simulink model "A2_live"  (R2024b)
settings: Solver=ode4  StartTime=0.0  StopTime=T_run  FixedStep=Ts_ctrl  RelTol=1e-3
values from neighbouring files (symbols this model uses):
  animate = 1    [A2_6_gps_setup.m]    (also in A2_gui_setup.m; A2_live_setup.m)
  R_LOS = evalin('base', 'R_LOS')    [A2_gui_report.m]
  Ts_ctrl = evalin('base', 'Ts_ctrl')    [A2_gui_report.m]
  u_ref = evalin('base', 'u_ref')    [A2_gui_report.m]
  wp_east = wp_ned(:,2).'    [A2_3_click_done.m]    (also in A2_3_click_todo.m; A2_6_gps_setup.m = [0   15   60   35]; A2_gui_report.m = evalin('base', 'wp_east'); A2_gui_setup.m = zeros(1, WP_MAX))
  wp_north = wp_ned(:,1).'    [A2_3_click_done.m]    (also in A2_3_click_todo.m; A2_6_gps_setup.m = [0   30   30   -5]; A2_gui_report.m = evalin('base', 'wp_north'); A2_gui_setup.m = zeros(1, WP_MAX))
  x0 = [0.1; 0; 0; 0; 0; psi_init]    [A2_6_gps_setup.m]    (also in A2_gui_setup.m = [0.1; 0; 0; 0; 0; 0]; A2_live_setup.m)
undefined symbols (not defined in the file or in its folder): beta_c, current_speed, Delta, F_max, F_plugin_max, guidance_mode, half_beam, k_prop, Kb, Kd_psi, Ki_u, Kp_psi, Kp_u, stop_hold, sw_mode, usv_p
libraries: slpidlib x1
settings Model: Creator=admin  LastModifiedBy=admin

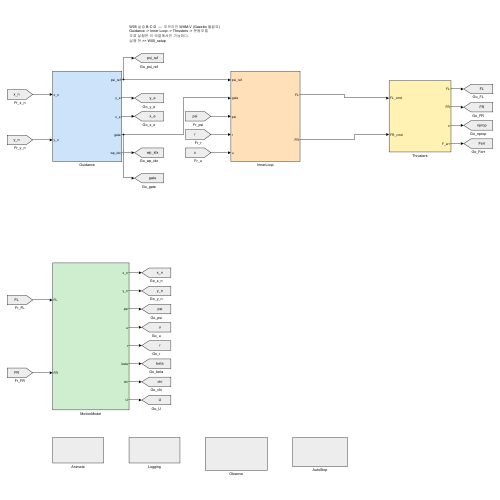
[thumbnail: Simulink's stored preview of the top-level diagram]
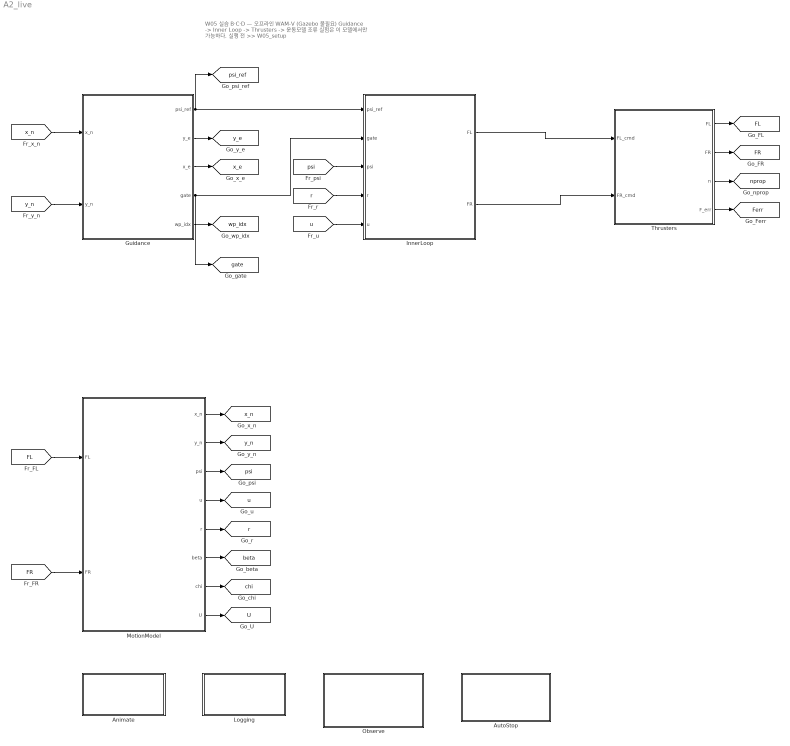
== system A2_live ==
  note: W05 실습 B·C·D  —  오프라인 WAM-V (Gazebo 불필요)
      | Guidance -> Inner Loop -> Thrusters -> 운동모델
      | 조류 실험은 이 모델에서만 가능하다.
      | 실행 전 >> W05_setup
  Animate : Subsystem
  AutoStop : Subsystem
  Guidance : Subsystem
  InnerLoop : Subsystem
  Logging : Subsystem
  MotionModel : Subsystem
  Observe : Subsystem
  Thrusters : Subsystem
  tag scope: FL=global, FR=global, Ferr=global, U=global, beta=global, chi=global, gate=global, nprop=global, psi=global, psi_ref=global, r=global, u=global, wp_idx=global, x_e=global, x_n=global, y_e=global, y_n=global
  wires:
  InnerLoop/2(FR) -> Thrusters/2(FR_cmd)
  InnerLoop/1(FL) -> Thrusters/1(FL_cmd)
  Guidance/4(gate) -> InnerLoop/2(gate), [gate]
  Guidance/1(psi_ref) -> InnerLoop/1(psi_ref), [psi_ref]
  Thrusters/1(FL) -> [FL]
  Thrusters/2(FR) -> [FR]
  Thrusters/3(n) -> [nprop]
  MotionModel/3(psi) -> [psi]
  MotionModel/5(r) -> [r]
  MotionModel/4(u) -> [u]
  MotionModel/1(x_n) -> [x_n]
  Guidance/2(y_e) -> [y_e]
  MotionModel/2(y_n) -> [y_n]
  [FL] -> MotionModel/1(FL)
  [FR] -> MotionModel/2(FR)
  [psi] -> InnerLoop/3(psi)
  [r] -> InnerLoop/4(r)
  [u] -> InnerLoop/5(u)
  [x_n] -> Guidance/1(x_n)
  [y_n] -> Guidance/2(y_n)
  Thrusters/4(F_err) -> [Ferr]
  MotionModel/8(U) -> [U]
  MotionModel/6(beta) -> [beta]
  MotionModel/7(chi) -> [chi]
  Guidance/3(x_e) -> [x_e]
  Guidance/5(wp_idx) -> [wp_idx]

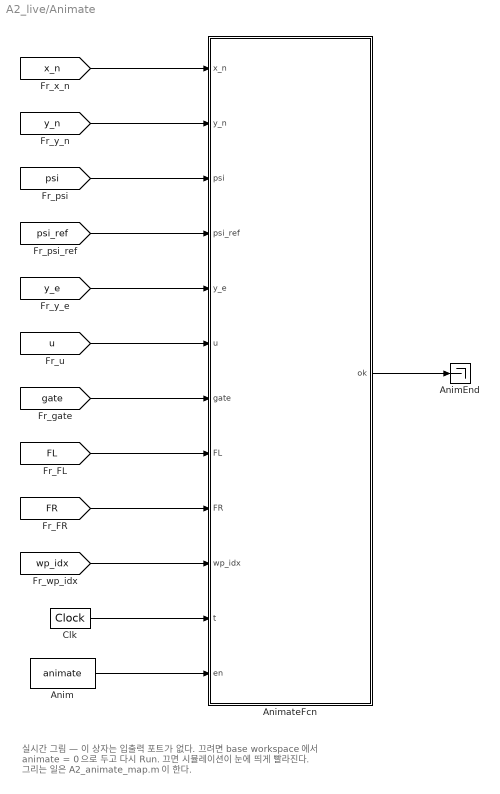
== system A2_live/Animate ==
  note: 실시간 그림 — 이 상자는 입출력 포트가 없다.
      | 끄려면 base workspace 에서  animate = 0  으로 두고 다시 Run.
      | 끄면 시뮬레이션이 눈에 띄게 빨라진다.
      | 그리는 일은 A2_animate_map.m 이 한다.
  Anim : Constant  Value=animate
  AnimEnd : Terminator
  AnimateFcn : MATLAB Function  TreatAsAtomicUnit=on
  Clk : DigitalClock  SampleTime=Ts_ctrl
  wires:
  [x_n] -> AnimateFcn/1(x_n)
  [y_n] -> AnimateFcn/2(y_n)
  [psi] -> AnimateFcn/3(psi)
  [psi_ref] -> AnimateFcn/4(psi_ref)
  [y_e] -> AnimateFcn/5(y_e)
  [u] -> AnimateFcn/6(u)
  [gate] -> AnimateFcn/7(gate)
  [FL] -> AnimateFcn/8(FL)
  [FR] -> AnimateFcn/9(FR)
  [wp_idx] -> AnimateFcn/10(wp_idx)
  Clk/1 -> AnimateFcn/11(t)
  Anim/1 -> AnimateFcn/12(en)
  AnimateFcn/1(ok) -> AnimEnd/1

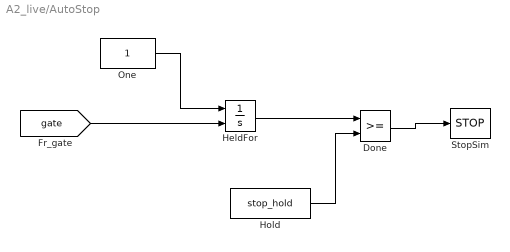
== system A2_live/AutoStop ==
  Done : RelationalOperator  OutDataTypeStr=boolean  RndMeth=Simplest  InputSameDT=off
  HeldFor : Integrator  ExternalReset=level
  Hold : Constant  Value=stop_hold
  One : Constant
  StopSim : Stop
  wires:
  One/1 -> HeldFor/1
  [gate] -> HeldFor/2
  HeldFor/1 -> Done/1
  Hold/1 -> Done/2
  Done/1 -> StopSim/1

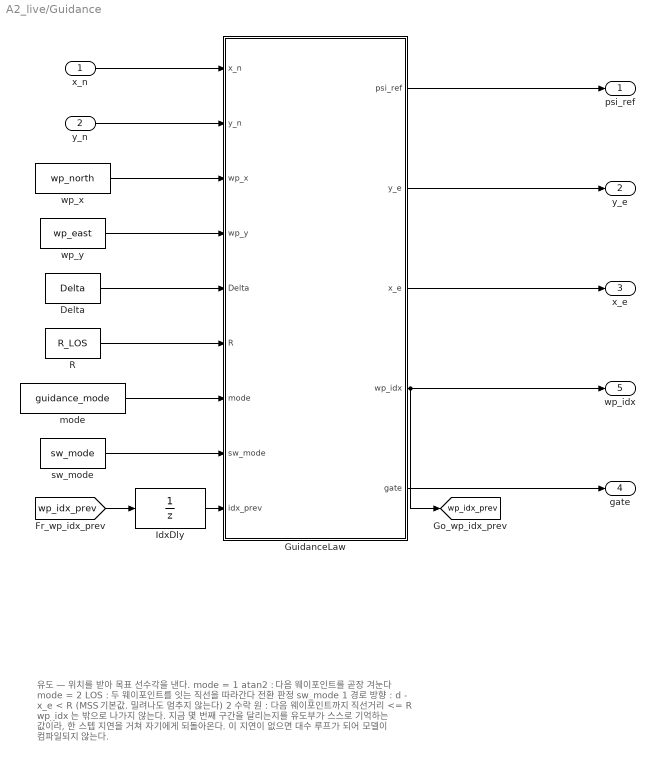
== system A2_live/Guidance ==
  note: 유도 — 위치를 받아 목표 선수각을 낸다.
      |   mode = 1  atan2 : 다음 웨이포인트를 곧장 겨눈다
      |   mode = 2  LOS   : 두 웨이포인트를 잇는 직선을 따라간다
      |
      | 전환 판정 sw_mode
      |   1  경로 방향 : d - x_e < R   (MSS 기본값. 밀려나도 멈추지 않는다)
      |   2  수락 원   : 다음 웨이포인트까지 직선거리 <= R
      |
      | wp_idx 는 밖으로 나가지 않는다. 지금 몇 번째 구간을 달리는지를
      | 유도부가 스스로 기억하는 값이라, 한 스텝 지연을 거쳐 자기에게 되돌아온다.
      | 이 지연이 없으면 대수 루프가 되어 모델이 컴파일되지 않는다.
  x_n : Inport
  y_n : Inport  Port=2
  Delta : Constant  Value=Delta
  GuidanceLaw : MATLAB Function  TreatAsAtomicUnit=on
  IdxDly : UnitDelay  Description=대수 루프 차단 + 사건 계수기 — 웨이포인트 번호는 정수이고, 유도부가 낸 값이 유도부로 되돌아온다. 미분방정식의 상태가 아니다.  InitialCondition=1  SampleTime=Ts_ctrl  HasFrameUpgradeWarning=on
  R : Constant  Value=R_LOS
  mode : Constant  Value=guidance_mode
  sw_mode : Constant  Value=sw_mode
  wp_x : Constant  Value=wp_north
  wp_y : Constant  Value=wp_east
  psi_ref : Outport
  y_e : Outport  Port=2
  x_e : Outport  Port=3
  gate : Outport  Port=4
  wp_idx : Outport  Port=5
  tag scope: wp_idx_prev=global
  wires:
  x_n/1 -> GuidanceLaw/1(x_n)
  y_n/1 -> GuidanceLaw/2(y_n)
  wp_x/1 -> GuidanceLaw/3(wp_x)
  wp_y/1 -> GuidanceLaw/4(wp_y)
  Delta/1 -> GuidanceLaw/5(Delta)
  R/1 -> GuidanceLaw/6(R)
  mode/1 -> GuidanceLaw/7(mode)
  sw_mode/1 -> GuidanceLaw/8(sw_mode)
  [wp_idx_prev] -> IdxDly/1
  IdxDly/1 -> GuidanceLaw/9(idx_prev)
  GuidanceLaw/1(psi_ref) -> psi_ref/1
  GuidanceLaw/2(y_e) -> y_e/1
  GuidanceLaw/3(x_e) -> x_e/1
  GuidanceLaw/5(gate) -> gate/1
  GuidanceLaw/4(wp_idx) -> wp_idx/1, [wp_idx_prev]

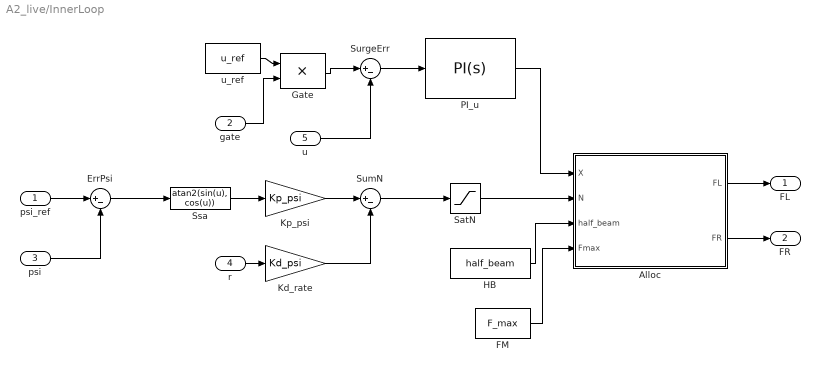
== system A2_live/InnerLoop ==
  psi_ref : Inport
  gate : Inport  Port=2
  psi : Inport  Port=3
  r : Inport  Port=4
  u : Inport  Port=5
  Alloc : MATLAB Function  TreatAsAtomicUnit=on
  ErrPsi : Sum  Inputs=|+-
  FM : Constant  Value=F_max
  Gate : Product
  HB : Constant  Value=half_beam
  Kd_rate : Gain  Gain=Kd_psi
  Kp_psi : Gain  Gain=Kp_psi
  PI_u : slpidlib/PID Controller  Controller=PI  Form=Parallel  TimeDomain=Continuous-time  UseExternalTs=off  SampleTime=-1  IntegratorMethod=Forward Euler  FilterMethod=Forward Euler  ControllerParametersSource=internal  P=Kp_u  I=Ki_u  UseKiTs=off  D=0  UseExternalDerivativeSource=off  N=100  UseFilter=on  TunerSelectOption=Transfer Function Based (PID Tuner App)  InitialConditionSource=internal  InitialConditionForIntegrator=0  InitialConditionForFilter=0  DifferentiatorICPrevScaledInput=0  ExternalReset=none  TrackingMode=off  Kt=1  LimitOutput=on  SatLimitsSource=internal  UpperSaturationLimit=2*F_max  LowerSaturationLimit=-2*F_max  LinearizeAsGain=on  AntiWindupMode=back-calculation  Kb=Kb  LimitIntegrator=off  UpperIntegratorSaturationLimit=inf  LowerIntegratorSaturationLimit=-inf  POutMin=[]  POutMax=[]  IOutMin=[]  IOutMax=[]  DOutMin=[]  DOutMax=[]  NOutMin=[]  NOutMax=[]  SumOutMin=[]  SumOutMax=[]  SaturationOutMin=[]  SaturationOutMax=[]  PParamMin=[]  PParamMax=[]  IParamMin=[]  IParamMax=[]  DParamMin=[]  DParamMax=[]  NParamMin=[]  NParamMax=[]  KbParamMin=[]  KbParamMax=[]  KtParamMin=[]  KtParamMax=[]  KbOutMin=[]  KbOutMax=[]  KtOutMin=[]  KtOutMax=[]  IntegratorOutMin=[]  IntegratorOutMax=[]  FilterOutMin=[]  FilterOutMax=[]  SumI1OutMin=[]  SumI1OutMax=[]  SumI2OutMin=[]  SumI2OutMax=[]  SumI3OutMin=[]  SumI3OutMax=[]  SumI4OutMin=[]  SumI4OutMax=[]  SumDOutMin=[]  SumDOutMax=[]  DifferentiatorOutMin=[]  DifferentiatorOutMax=[]  FilterDiffOutCoefMin=[]  FilterDiffOutCoefMax=[]  ReciprocalOutMin=[]  ReciprocalOutMax=[]  SumDenOutMin=[]  SumDenOutMax=[]  SumNumOutMin=[]  SumNumOutMax=[]  DivideOutMin=[]  DivideOutMax=[]  UdiffTsProdOutMin=[]  UdiffTsProdOutMax=[]  NTsProdOutMin=[]  NTsProdOutMax=[]  UintegralTsProdOutMin=[]  UintegralTsProdOutMax=[]  UngainTsProdOutMin=[]  UngainTsProdOutMax=[]  ClampingZeroOutDataTypeStr=Inherit: Inherit via back propagation  ClampingZeroOutMin=[]  ClampingZeroOutMax=[]  FilterDenConstantOutDataTypeStr=Inherit: Inherit via back propagation  FilterDenConstantOutMin=[]  FilterDenConstantOutMax=[]  PCopyOutDataTypeStr=Inherit: Inherit via back propagation  PCopyOutMin=[]  PCopyOutMax=[]  NCopyOutDataTypeStr=Inherit: Inherit via back propagation  NCopyOutMin=[]  NCopyOutMax=[]  IntegratorContinuousStateAttributes=''  IntegratorStateMustResolveToSignalObject=off  IntegratorRTWStateStorageClass=Auto  FilterContinuousStateAttributes=''  FilterStateMustResolveToSignalObject=off  FilterRTWStateStorageClass=Auto  ParallelPVariant=InternalParameters  IdealPVariant=Disabled  IVariant=InternalParameters  DVariant=Disabled  IntegratorVariant=Continuous  SatVariant=Enabled  AWVariant=BackCalculation  PCopyVariant=Disabled  TRVariant=Disabled  FdbkBlocksVariant=Forward  IdealPFdbkVariant=Disabled  SatFdbkVariant=Disabled  DerivativeFilterVariant=Disabled  NVariant=Disabled  NCopyVariant=Disabled_SignalSpec  FilterICVariant=Disabled  IntegratorICVariant=InternalICs  ExternalResetVariant=Disabled  TRSumVariant=Passthrough  SumFdbkVariant=Disabled  SumVariant=Sum_PI  TsampFilterVariant=InternalTs  TsampNgainVariant=Passthrough  TsampIntegralVariant=Disabled_SignalSpec  ExternalSaturationOutDataTypeStr=Inherit: Same as second input  DerivativeSourceVariant=Disabled  PreIntVariant=InternalPreInt
  SatN : Saturate  UpperLimit=2*F_max*half_beam  LowerLimit=-2*F_max*half_beam
  Ssa : Fcn  Expr=atan2(sin(u), cos(u))
  SumN : Sum  Inputs=|+-
  SurgeErr : Sum  Inputs=|+-
  u_ref : Constant  Value=u_ref
  FL : Outport
  FR : Outport  Port=2
  wires:
  ErrPsi/1 -> Ssa/1
  u_ref/1 -> Gate/1
  psi_ref/1 -> ErrPsi/1
  psi/1 -> ErrPsi/2
  gate/1 -> Gate/2
  Ssa/1 -> Kp_psi/1
  Alloc/1(FL) -> FL/1
  Gate/1 -> SurgeErr/1
  r/1 -> Kd_rate/1
  u/1 -> SurgeErr/2
  Kp_psi/1 -> SumN/1
  Kd_rate/1 -> SumN/2
  SurgeErr/1 -> PI_u/1
  SumN/1 -> SatN/1
  PI_u/1 -> Alloc/1(X)
  SatN/1 -> Alloc/2(N)
  HB/1 -> Alloc/3(half_beam)
  FM/1 -> Alloc/4(Fmax)
  Alloc/2(FR) -> FR/1

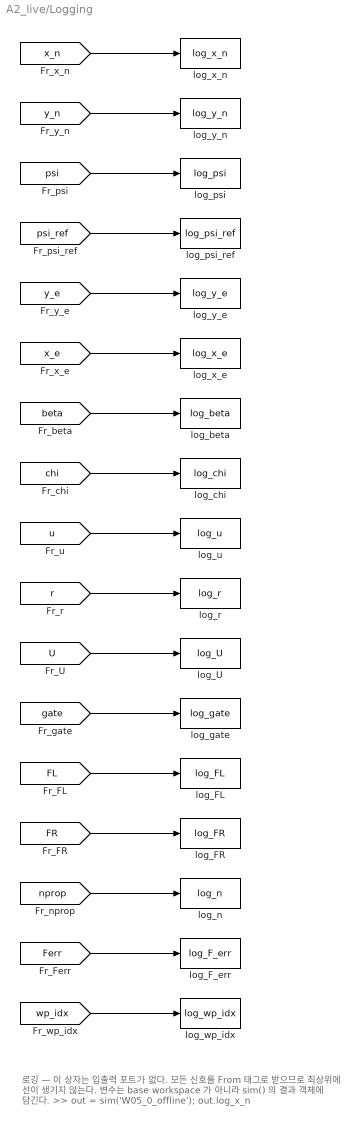
== system A2_live/Logging ==
  note: 로깅 — 이 상자는 입출력 포트가 없다.
      | 모든 신호를 From 태그로 받으므로 최상위에 선이 생기지 않는다.
      | 변수는 base workspace 가 아니라 sim() 의 결과 객체에 담긴다.
      |   >> out = sim('W05_0_offline');  out.log_x_n
  log_FL : ToWorkspace  VariableName=log_FL  SaveFormat=Timeseries  SampleTime=Ts_ctrl
  log_FR : ToWorkspace  VariableName=log_FR  SaveFormat=Timeseries  SampleTime=Ts_ctrl
  log_F_err : ToWorkspace  VariableName=log_F_err  SaveFormat=Timeseries  SampleTime=Ts_ctrl
  log_U : ToWorkspace  VariableName=log_U  SaveFormat=Timeseries  SampleTime=Ts_ctrl
  log_beta : ToWorkspace  VariableName=log_beta  SaveFormat=Timeseries  SampleTime=Ts_ctrl
  log_chi : ToWorkspace  VariableName=log_chi  SaveFormat=Timeseries  SampleTime=Ts_ctrl
  log_gate : ToWorkspace  VariableName=log_gate  SaveFormat=Timeseries  SampleTime=Ts_ctrl
  log_n : ToWorkspace  VariableName=log_n  SaveFormat=Timeseries  SampleTime=Ts_ctrl
  log_psi : ToWorkspace  VariableName=log_psi  SaveFormat=Timeseries  SampleTime=Ts_ctrl
  log_psi_ref : ToWorkspace  VariableName=log_psi_ref  SaveFormat=Timeseries  SampleTime=Ts_ctrl
  log_r : ToWorkspace  VariableName=log_r  SaveFormat=Timeseries  SampleTime=Ts_ctrl
  log_u : ToWorkspace  VariableName=log_u  SaveFormat=Timeseries  SampleTime=Ts_ctrl
  log_wp_idx : ToWorkspace  VariableName=log_wp_idx  SaveFormat=Timeseries  SampleTime=Ts_ctrl
  log_x_e : ToWorkspace  VariableName=log_x_e  SaveFormat=Timeseries  SampleTime=Ts_ctrl
  log_x_n : ToWorkspace  VariableName=log_x_n  SaveFormat=Timeseries  SampleTime=Ts_ctrl
  log_y_e : ToWorkspace  VariableName=log_y_e  SaveFormat=Timeseries  SampleTime=Ts_ctrl
  log_y_n : ToWorkspace  VariableName=log_y_n  SaveFormat=Timeseries  SampleTime=Ts_ctrl
  wires:
  [x_n] -> log_x_n/1
  [y_n] -> log_y_n/1
  [psi] -> log_psi/1
  [psi_ref] -> log_psi_ref/1
  [y_e] -> log_y_e/1
  [x_e] -> log_x_e/1
  [beta] -> log_beta/1
  [chi] -> log_chi/1
  [u] -> log_u/1
  [r] -> log_r/1
  [U] -> log_U/1
  [gate] -> log_gate/1
  [FL] -> log_FL/1
  [FR] -> log_FR/1
  [nprop] -> log_n/1
  [Ferr] -> log_F_err/1
  [wp_idx] -> log_wp_idx/1

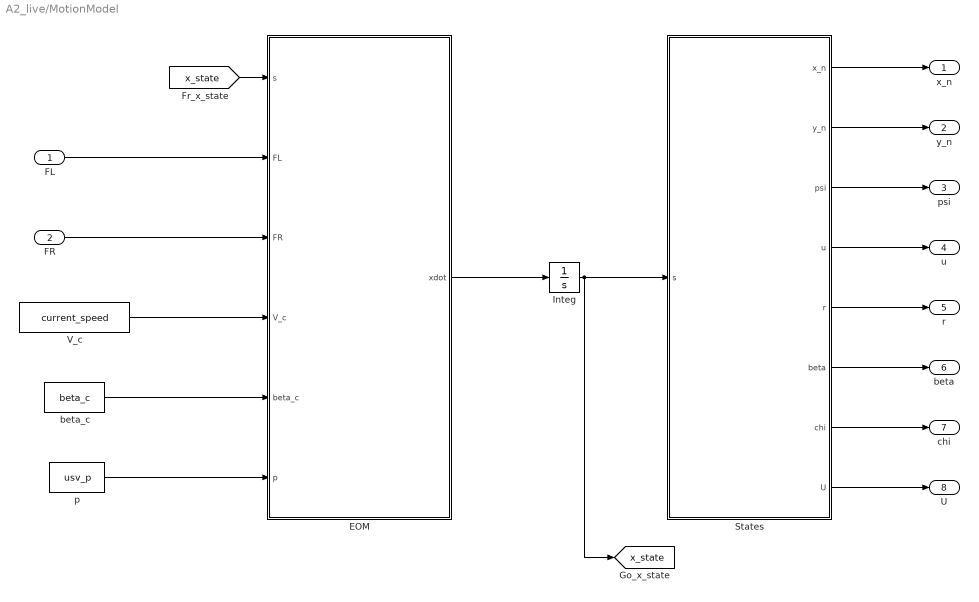
== system A2_live/MotionModel ==
  FL : Inport
  FR : Inport  Port=2
  EOM : MATLAB Function  TreatAsAtomicUnit=on
  Integ : Integrator  InitialCondition=x0
  States : MATLAB Function  TreatAsAtomicUnit=on
  V_c : Constant  Value=current_speed
  beta_c : Constant  Value=beta_c
  p : Constant  Value=usv_p
  x_n : Outport
  y_n : Outport  Port=2
  psi : Outport  Port=3
  u : Outport  Port=4
  r : Outport  Port=5
  beta : Outport  Port=6
  chi : Outport  Port=7
  U : Outport  Port=8
  tag scope: x_state=global
  wires:
  FL/1 -> EOM/2(FL)
  FR/1 -> EOM/3(FR)
  V_c/1 -> EOM/4(V_c)
  beta_c/1 -> EOM/5(beta_c)
  p/1 -> EOM/6(p)
  EOM/1(xdot) -> Integ/1
  Integ/1 -> States/1(s), [x_state]
  [x_state] -> EOM/1(s)
  States/1(x_n) -> x_n/1
  States/2(y_n) -> y_n/1
  States/3(psi) -> psi/1
  States/4(u) -> u/1
  States/5(r) -> r/1
  States/6(beta) -> beta/1
  States/7(chi) -> chi/1
  States/8(U) -> U/1

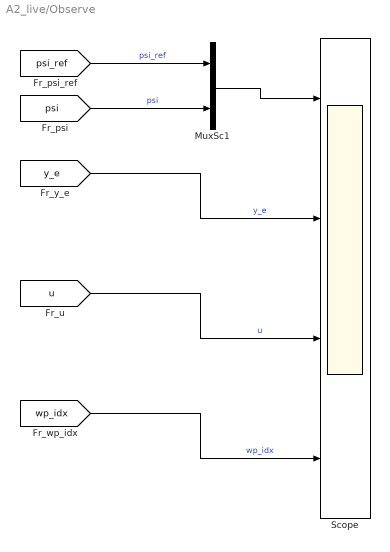
== system A2_live/Observe ==
  MuxSc1 : Mux  Inputs=2
  Scope : Scope  NumInputPorts=4
  wires:
  [psi_ref] -> MuxSc1/1  "psi_ref"
  [psi] -> MuxSc1/2  "psi"
  MuxSc1/1 -> Scope/1
  [y_e] -> Scope/2  "y_e"
  [u] -> Scope/3  "u"
  [wp_idx] -> Scope/4  "wp_idx"

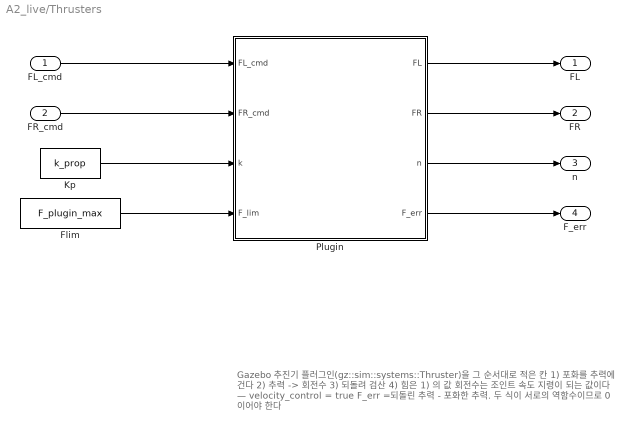
== system A2_live/Thrusters ==
  note: Gazebo 추진기 플러그인(gz::sim::systems::Thruster)을 그 순서대로 적은 칸
      | 1) 포화를 추력에 건다  2) 추력 -> 회전수  3) 되돌려 검산  4) 힘은 1) 의 값
      | 회전수는 조인트 속도 지령이 되는 값이다 — velocity_control = true
      | F_err = 되돌린 추력 - 포화한 추력. 두 식이 서로의 역함수이므로 0 이어야 한다
  FL_cmd : Inport
  FR_cmd : Inport  Port=2
  Flim : Constant  Value=F_plugin_max
  Kp : Constant  Value=k_prop
  Plugin : MATLAB Function  TreatAsAtomicUnit=on
  FL : Outport
  FR : Outport  Port=2
  n : Outport  Port=3
  F_err : Outport  Port=4
  wires:
  FL_cmd/1 -> Plugin/1(FL_cmd)
  Plugin/1(FL) -> FL/1
  FR_cmd/1 -> Plugin/2(FR_cmd)
  Plugin/2(FR) -> FR/1
  Kp/1 -> Plugin/3(k)
  Plugin/3(n) -> n/1
  Flim/1 -> Plugin/4(F_lim)
  Plugin/4(F_err) -> F_err/1

== matlab function A2_live/InnerLoop/Alloc ==
  data: X input; FL output; N input; half_beam input; Fmax input; FR output
function [FL, FR] = Alloc(X, N, half_beam, Fmax)
%#codegen
% Differential thrust allocation for two aft thrusters.
%   X = FL + FR              surge force [N]
%   N = (FL - FR)*half_beam  yaw moment  [N*m]
FL = X/2 + N/(2*half_beam);
FR = X/2 - N/(2*half_beam);
if FL >  Fmax, FL =  Fmax; end
if FL < -Fmax, FL = -Fmax; end
if FR >  Fmax, FR =  Fmax; end
if FR < -Fmax, FR = -Fmax; end

== matlab function A2_live/Guidance/GuidanceLaw ==
  data: x_n input; psi_ref output; y_n input; wp_x input; wp_y input; Delta input; R input; mode input; sw_mode input; idx_prev input; y_e output; x_e output; wp_idx output; gate output
function [psi_ref, y_e, x_e, wp_idx, gate] = GuidanceLaw(x_n, y_n, wp_x, wp_y, Delta, R, mode, sw_mode, idx_prev)
%#codegen
% Waypoint guidance. Two laws in one block. Both return a HEADING command,
% following the MSS demo demoOtterUSVHeadingControl.slx and GNC/LOSchi.m.
%   mode 1 = atan2 : aim straight at the next waypoint (point chasing)
%   mode 2 = LOS   : follow the straight line between two waypoints
% Switching criterion (sw_mode):
%   1 = along-track : d - x_e < R      (MSS / Fossen default, cannot hang)
%   2 = circle      : distance to the next waypoint <= R

n = numel(wp_x);
k = min(max(idx_prev, 1), n-1);        % index of the active leg

xk  = wp_x(k);    yk  = wp_y(k);       % leg start
xk1 = wp_x(k+1);  yk1 = wp_y(k+1);     % leg end = next waypoint

% path-tangential angle of the active leg, measured from North
pi_p = atan2(yk1 - yk, xk1 - xk);

% Both errors come out of ONE rotation of (p - p_k) into the path frame.
% x_e = how far ALONG the leg,  y_e = how far TO THE SIDE of it.
% Computed the same way for BOTH guidance laws so that the two can be
% compared with the same yardstick.
x_e =  (x_n - xk)*cos(pi_p) + (y_n - yk)*sin(pi_p);
y_e = -(x_n - xk)*sin(pi_p) + (y_n - yk)*cos(pi_p);

if mode == 1
    psi_ref = atan2(yk1 - y_n, xk1 - x_n);
else
    psi_ref = pi_p - atan(y_e / Delta);
end

% --- waypoint switching ---------------------------------------------
% d is the leg length, so d - x_e is the along-track distance REMAINING.
% The circle test is always the stricter of the two, because
%     distance = sqrt((d - x_e)^2 + y_e^2) >= d - x_e
% A boat blown wide of a waypoint never enters that circle, and a mission
% that waits for it waits for ever. The along-track test cannot hang.
d = sqrt((xk1 - xk)^2 + (yk1 - yk)^2);
if sw_mode == 1
    reached = (d - x_e) < R;
else
    reached = sqrt((xk1 - x_n)^2 + (yk1 - y_n)^2) <= R;
end

% wp_idx = n means "mission finished" and it LATCHES: once the last leg is
% done, the boat stays stopped even if the current pushes it back behind the
% finish line (then reached would turn false again).
if idx_prev >= n
    wp_idx = n;                         % already finished - stay finished
elseif reached && (k < n-1)
    wp_idx = k + 1;
elseif reached && (k == n-1)
    wp_idx = n;                         % last leg done
else
    wp_idx = k;
end

% gate = 0 brings the boat to a stop. Without it the boat would follow the
% last leg forever.
gate = double(wp_idx < n);

== matlab function A2_live/Thrusters/Plugin ==
  data: FL_cmd input; FL output; FR_cmd input; k input; F_lim input; FR output; n output; F_err output
function [FL, FR, n, F_err] = Plugin(FL_cmd, FR_cmd, k, F_lim)
%#codegen
% Gazebo 추진기 플러그인이 하는 일을 소스와 같은 순서로 적는다.
%   gz-sim7  src/systems/thruster/Thruster.cc

% 1) 포화 — 플러그인은 **추력에** 건다 (OnCmdThrust, :520-521)
%      thrust = clamp(cmd, cmdMin, cmdMax),  cmdMax = max_thrust_cmd
F = [FL_cmd; FR_cmd];
F = max(-F_lim, min(F_lim, F));

% 2) 추력 -> 회전수 (ThrustToAngularVec, :562-584). 이 값이 조인트
%    속도 지령이 된다 — velocity_control = true (:740-756)
%      omega = sign(F*Ct)*sqrt(|F|/(rho*Ct*D^4)),  k = rho*Ct*D^4
%    Ct > 0 이므로 sign(F*Ct) = sign(F) 다
n = sign(F) .* sqrt(abs(F)/k);

% 3) 회전수 -> 추력 (AngularVelToThrust, :593-599). 플러그인에서는
%    회전수 지령 모드에만 쓰인다. 여기서는 2) 를 되돌려 맞는지 보는
%    **검산**이다 — 두 식이 서로의 역함수이므로 0 이 나와야 한다
%      F = rho*Ct*D^4 * |omega| * omega
F_chk = k * abs(n) .* n;
F_err = F_chk - F;

% 4) 링크에 가는 힘은 되돌린 값이 아니라 포화만 거친 지령이다
%    (AddWorldWrench 가 desiredThrust 를 그대로 쓴다, :770-773)
FL = F(1);
FR = F(2);

== matlab function A2_live/MotionModel/EOM ==
  data: s input; xdot output; FL input; FR input; V_c input; beta_c input; p input
function xdot = EOM(s, FL, FR, V_c, beta_c, p)
%#codegen
% 3-DOF WAM-V equations of motion, NED.
% Coefficients come straight from the Gazebo VRX plugins:
%   drag       : SimpleHydrodynamics  (Xu Xuu Yv Yvv Nr Nrr)
%   mass       : wamv_base.urdf.xacro (180 kg hull + engines)
%   added mass : zero in VRX (xDotU = yDotV = nDotR = 0)
% Ocean current exists only here. Gazebo has no current plugin.
%   s = [u v r N E psi]'
%   p = [m Izz Xu Xuu Yv Yvv Nr Nrr half_beam]'

u = s(1); v = s(2); r = s(3); psi = s(6);
m=p(1); Izz=p(2); Xu=p(3); Xuu=p(4); Yv=p(5); Yvv=p(6);
Nr=p(7); Nrr=p(8); b_half=p(9);

% current in the body frame -> velocity relative to the water
u_c = V_c*cos(beta_c - psi);
v_c = V_c*sin(beta_c - psi);
u_r = u - u_c;
v_r = v - v_c;

% differential thrust -> surge force and yaw moment
X = FL + FR;
N = (FL - FR)*b_half;

% drag acts on the velocity relative to the water
Dx = (Xu + Xuu*abs(u_r))*u_r;
Dy = (Yv + Yvv*abs(v_r))*v_r;
Dn = (Nr + Nrr*abs(r))*r;

du = (X - Dx)/m + v*r;      % rigid-body Coriolis
dv = (  - Dy)/m - u*r;
dr = (N - Dn)/Izz;

xdot = [du; dv; dr;
        u*cos(psi) - v*sin(psi);   % kinematics use absolute velocity
        u*sin(psi) + v*cos(psi);
        r];

== matlab function A2_live/MotionModel/States ==
  data: s input; x_n output; y_n output; psi output; u output; r output; beta output; chi output; U output
function [x_n, y_n, psi, u, r, beta, chi, U] = States(s)
%#codegen
% Pick the navigation quantities out of the state vector.
% In the VRX model this job is done by the Nav block,
% which also has to convert ENU to NED.
u = s(1); v = s(2); r = s(3);
x_n = s(4); y_n = s(5); psi = s(6);
U    = sqrt(u*u + v*v);      % speed over ground
beta = atan2(v, u);          % crab angle
c    = psi + beta;           % course angle
chi  = atan2(sin(c), cos(c));

== matlab function A2_live/Animate/AnimateFcn ==
  data: x_n input; y_n input; psi input; psi_ref input; y_e input; u input; ok output; gate input; FL input; FR input; wp_idx input; t input; en input
function ok = AnimateFcn(x_n, y_n, psi, psi_ref, y_e, u, gate, FL, FR, wp_idx, t, en)
%#codegen
% Live plot while the model runs. A MATLAB Function block cannot
% plot, so the drawing function is declared extrinsic: Simulink
% calls plain MATLAB instead of generating code for it.
coder.extrinsic('A2_animate_map');
ok = 1;
if en > 0.5
    A2_animate_map(x_n, y_n, psi, psi_ref, y_e, u, gate, FL, FR, wp_idx, t);
end
